simulink model "ACC4_FFNN_trainoss_30_30_30_ep_100_Nor_20250528"  (R2021a)
settings: Solver=FixedStepAuto  StartTime=0.0  StopTime=T  RelTol=1e-3
undefined symbols (not defined in the file or in its folder): t_gap, Ts, v0_ego, v0_lead, v_set, x0_ego, x0_lead, x_gain, x_offset, y_gain, y_offset
libraries: neural x95
(part 5 of 5)

== system ACC4_FFNN_trainoss_30_30_30_ep_100_Nor_20250528/Feed-Forward Neural Network/Layer 4/Delays 1 ==
  "p{4}" : Inport  PortDimensions=30
      mask Display: e = 0.06;c1 = [120 230 180]/255;c2 = ([120 230 180]+0)/(256+128);c3 = ([120 230 180]+128)/(256+128);patch([0 1 1 0],[0 0 1 1],c1);patch([0 1 1 1-e 1-e 0+e],[0 0 1 1-e 0+e 0+e],c2);patch([0 0 1 1-e 0+e 0+e],[0 1 1 1-e 1-e 0+e],c3);plot([0 1 1 0 0],[0 0 1 1 0]);
  mux : Mux  Inputs=1
      mask Display: e = 0.06;c1 = [120 150 230]/255;c2 = ([120 150 230]+0)/383;c3 = ([120 150 230]+128)/383;patch([0 1 1 0],[0 0 1 1],c1);patch([0 1 1 1-e 1-e 0+e],[0 0 1 1-e 0+e 0+e],c2);patch([0 0 1 1-e 0+e 0+e],[0 1 1 1-e 1-e 0+e],c3);plot([0 1 1 0 0],[0 0 1 1 0]);disp('Mux')
  "pd{4,3}" : Outport
      mask Display: e = 0.06;c1 = [120 230 180]/255;c2 = ([120 230 180]+0)/(256+128);c3 = ([120 230 180]+128)/(256+128);patch([0 1 1 0],[0 0 1 1],c1);patch([0 1 1 1-e 1-e 0+e],[0 0 1 1-e 0+e 0+e],c2);patch([0 0 1 1-e 0+e 0+e],[0 1 1 1-e 1-e 0+e],c3);plot([0 1 1 0 0],[0 0 1 1 0]);
  wires:
  mux/1 -> "pd{4,3}"/1
  "p{4}"/1 -> mux/1

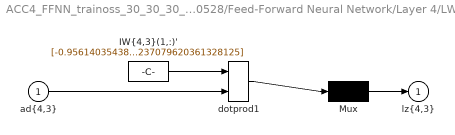
== system ACC4_FFNN_trainoss_30_30_30_ep_100_Nor_20250528/Feed-Forward Neural Network/Layer 4/LW{4,3} ==
  "ad{4,3}" : Inport  PortDimensions=30
      mask Display: e = 0.06;c1 = [120 230 180]/255;c2 = ([120 230 180]+0)/(256+128);c3 = ([120 230 180]+128)/(256+128);patch([0 1 1 0],[0 0 1 1],c1);patch([0 1 1 1-e 1-e 0+e],[0 0 1 1-e 0+e 0+e],c2);patch([0 0 1 1-e 0+e 0+e],[0 1 1 1-e 1-e 0+e],c3);plot([0 1 1 0 0],[0 0 1 1 0]);
  "IW{4,3}(1,:)'" : Constant  Value=[-0.95614035438404254563238282571546733379364013671875;0.6362019048678677624053534600534476339817047119140625;-0.6415809984175366853520472432137466967105865478515625;-0.668581820268475013335773837752640247344970703125;-0.62411868107123946725067753504845313727855682373046875;0.38149429431920733879479712413740344345569610595703125;-0.5858444465497070208215291131637059152126312255859375;-0.35367625429934024250400170785724185407161712646484375;0.5366702941194920750689334454364143311977386474609375;0.0023001892920386790564180046203546226024627685546875;0.79289017592470767414880583601188845932483673095703125;-0.884293745925841978561265932512469589710235595703125;-0.0916896029225741371337932150709093548357486724853515625;0.144493120967094046402934282014030031859874725341796875;0.13013431955435716957936165272258222103118896484375;0.633231310324929186350573218078352510929107666015625;-0.72232487491139274471407816236023791134357452392578125;-0.39933339676576584675871117724454961717128753662109375;-1.02107800114900282295593569870106875896453857421875;0.9022147157805451289647180601605214178562164306640625;0.5416004903041280460485040748608298599720001220703125;0.499098851860260206425579099231981672346591949462890625;-0.72227032571813065686683330568484961986541748046875;-0.29406487632623379280261133317253552377223968505859375;-0.673343240725825520343050811788998544216156005859375;-0.0022217314583966147299720628183195003657601773738861083984375;0.6176554685366379970901107299141585826873779296875;0.277801086906872607418250709088169969618320465087890625;0.33160538792325178203412860966636799275875091552734375;0.30345661145186142437779608371783979237079620361328125]
      mask Display: e = 0.06;c1 = [120 150 230]/255;c2 = ([120 150 230]+0)/383;c3 = ([120 150 230]+128)/383;patch([0 1 1 0],[0 0 1 1],c1);patch([0 1 1 1-e 1-e 0+e],[0 0 1 1-e 0+e 0+e],c2);patch([0 0 1 1-e 0+e 0+e],[0 1 1 1-e 1-e 0+e],c3);plot([0 1 1 0 0],[0 0 1 1 0]);disp('weights');
  Mux : Mux  Inputs=1
      mask Display: e = 0.06;c1 = [120 150 230]/255;c2 = ([120 150 230]+0)/383;c3 = ([120 150 230]+128)/383;patch([0 1 1 0],[0 0 1 1],c1);patch([0 1 1 1-e 1-e 0+e],[0 0 1 1-e 0+e 0+e],c2);patch([0 0 1 1-e 0+e 0+e],[0 1 1 1-e 1-e 0+e],c3);plot([0 1 1 0 0],[0 0 1 1 0]);disp('Mux');
  dotprod1 : neural/Weight Functions/dotprod
  "lz{4,3}" : Outport
      mask Display: e = 0.06;c1 = [120 230 180]/255;c2 = ([120 230 180]+0)/(256+128);c3 = ([120 230 180]+128)/(256+128);patch([0 1 1 0],[0 0 1 1],c1);patch([0 1 1 1-e 1-e 0+e],[0 0 1 1-e 0+e 0+e],c2);patch([0 0 1 1-e 0+e 0+e],[0 1 1 1-e 1-e 0+e],c3);plot([0 1 1 0 0],[0 0 1 1 0]);
  wires:
  Mux/1 -> "lz{4,3}"/1
  dotprod1/1 -> Mux/1
  "ad{4,3}"/1 -> dotprod1/2
  "IW{4,3}(1,:)'"/1 -> dotprod1/1
